simulink model "three_leg_switched"  (R2025b)
settings: Solver=FixedStepDiscrete  StartTime=0.0  StopTime=Tstop  FixedStep=Ts  RelTol=1e-3
values from neighbouring files (symbols this model uses):
  C = case_params(S, phase_deg, strcmp(policy, 'plan'), td_us, Ts)    [run_case.m]
  Tsw = C.Tsw    [ctrl_step.m]
undefined symbols (not defined in the file or in its folder): Ts
libraries: fl_lib x9, nesl_utility x8, ee_lib x6
settings Model: Creator=Asus ROG Strix G16  LastModifiedBy=Asus ROG Strix G16
settings DataIOCC: SaveOutput=off  SignalLogging=off  SaveTime=off

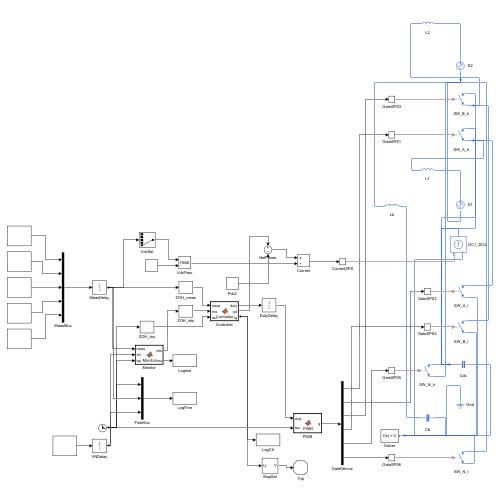
[thumbnail: Simulink's stored preview of the top-level diagram]
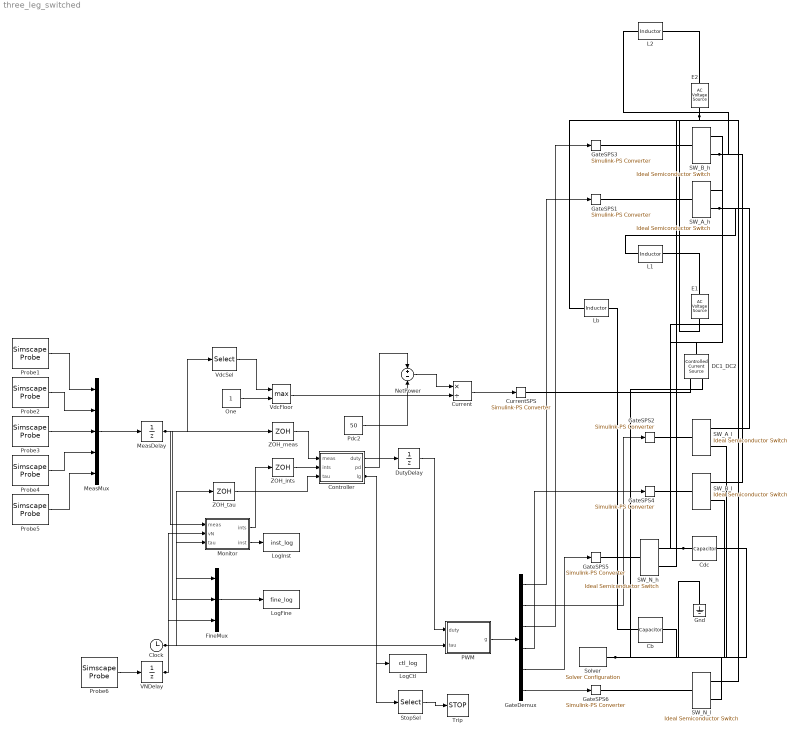
== system three_leg_switched ==
  Cb : fl_lib/Electrical/Electrical Elements/Capacitor  c=0.00025000000000000001 F  r=0 Ohm  g=0 1/Ohm  i_specify=off  i_priority=None  i=0 A  i_nominal_specify=off  i_nominal_value=1  i_nominal_unit=A  v_specify=off  v_priority=None  v=0 V  v_nominal_specify=off  v_nominal_value=1  v_nominal_unit=V  vc_specify=on  vc_priority=High  vc=C.vb0 V  vc_nominal_specify=off  vc_nominal_value=1  vc_nominal_unit=V
  Cdc : fl_lib/Electrical/Electrical Elements/Capacitor  c=2.0000000000000002e-05 F  r=0 Ohm  g=0 1/Ohm  i_specify=off  i_priority=None  i=0 A  i_nominal_specify=off  i_nominal_value=1  i_nominal_unit=A  v_specify=off  v_priority=None  v=0 V  v_nominal_specify=off  v_nominal_value=1  v_nominal_unit=V  vc_specify=on  vc_priority=High  vc=C.Vdc0 V  vc_nominal_specify=off  vc_nominal_value=1  vc_nominal_unit=V
  Clock : Clock
  Controller : MATLAB Function  TreatAsAtomicUnit=on
  Current : Product  Inputs=*/
  CurrentSPS : nesl_utility/Simulink-PS Converter  PhysicalDomain=network_engine_domain  SubClassName=ps_input  LeftPortType=input  RightPortType=output  PseudoPeriodic=off  Frequencies=[]  NoiseDistribution=none  NoiseParameters=[]  Unit=1  AffineConversion=off  FilteringAndDerivatives=provide  SimscapeFilterOrder=1  InputFilterTimeConstant=0.001  UdotUserProvided=0
  DC1_DC2 : fl_lib/Electrical/Electrical Sources/Controlled Current Source
  DutyDelay : UnitDelay  InitialCondition=C.duty0  SampleTime=Tsw  HasFrameUpgradeWarning=on
  E1 : fl_lib/Electrical/Electrical Sources/AC Voltage Source  amp=80 V  shift=C.theta0_deg deg  frequency=50 Hz
  E2 : fl_lib/Electrical/Electrical Sources/AC Voltage Source  amp=80 V  shift=C.theta0_deg + 0 deg  frequency=50 Hz
  FineMux : Mux  Inputs=3
  GateDemux : Demux  Outputs=6
  GateSPS{1..6} (6 alike) : nesl_utility/Simulink-PS Converter  PhysicalDomain=network_engine_domain  SubClassName=ps_input  LeftPortType=input  RightPortType=output  PseudoPeriodic=off  Frequencies=[]  NoiseDistribution=none  NoiseParameters=[]  Unit=1  AffineConversion=off  FilteringAndDerivatives=provide  SimscapeFilterOrder=1  InputFilterTimeConstant=0.001  UdotUserProvided=0
  Gnd : fl_lib/Electrical/Electrical Elements/Electrical Reference
  L1 : fl_lib/Electrical/Electrical Elements/Inductor  l=0.002 H  r=0.10000000000000001 Ohm  g=1e-9 1/Ohm  i_specify=off  i_priority=None  i=0 A  i_nominal_specify=off  i_nominal_value=1  i_nominal_unit=A  v_specify=off  v_priority=None  v=0 V  v_nominal_specify=off  v_nominal_value=1  v_nominal_unit=V  i_L_specify=on  i_L_priority=High  i_L=C.i10 A  i_L_nominal_specify=off  i_L_nominal_value=1  i_L_nominal_unit=A
  L2 : fl_lib/Electrical/Electrical Elements/Inductor  l=0.002 H  r=0.10000000000000001 Ohm  g=1e-9 1/Ohm  i_specify=off  i_priority=None  i=0 A  i_nominal_specify=off  i_nominal_value=1  i_nominal_unit=A  v_specify=off  v_priority=None  v=0 V  v_nominal_specify=off  v_nominal_value=1  v_nominal_unit=V  i_L_specify=on  i_L_priority=High  i_L=C.i20 A  i_L_nominal_specify=off  i_L_nominal_value=1  i_L_nominal_unit=A
  Lb : fl_lib/Electrical/Electrical Elements/Inductor  l=0.001 H  r=0.10000000000000001 Ohm  g=1e-9 1/Ohm  i_specify=off  i_priority=None  i=0 A  i_nominal_specify=off  i_nominal_value=1  i_nominal_unit=A  v_specify=off  v_priority=None  v=0 V  v_nominal_specify=off  v_nominal_value=1  v_nominal_unit=V  i_L_specify=on  i_L_priority=High  i_L=C.ib0 A  i_L_nominal_specify=off  i_L_nominal_value=1  i_L_nominal_unit=A
  LogCtl : ToWorkspace  VariableName=ctl_log  SampleTime=-1
  LogFine : ToWorkspace  VariableName=fine_log  SampleTime=-1
      settings: Decimation=fine_dec
  LogInst : ToWorkspace  VariableName=inst_log  SampleTime=-1
      settings: MaxDataPoints=1
  MeasDelay : UnitDelay  InitialCondition=C.meas0  SampleTime=Ts  HasFrameUpgradeWarning=on
  MeasMux : Mux  Inputs=5
  Monitor : MATLAB Function  TreatAsAtomicUnit=on
  NetPower : Sum  Inputs=+-
  One : Constant
  PWM : MATLAB Function  TreatAsAtomicUnit=on
  Pdc2 : Constant  Value=50
  Probe1 : SimscapeProbe  BoundBlock=7  Variables="{\"i_L\":{\"Probing\":\"ON\"}}"
  Probe2 : SimscapeProbe  BoundBlock=8  Variables="{\"i_L\":{\"Probing\":\"ON\"}}"
  Probe3 : SimscapeProbe  BoundBlock=6  Variables="{\"i_L\":{\"Probing\":\"ON\"}}"
  Probe4 : SimscapeProbe  BoundBlock=5  Variables="{\"vc\":{\"Probing\":\"ON\"}}"
  Probe5 : SimscapeProbe  BoundBlock=3  Variables="{\"vc\":{\"Probing\":\"ON\"}}"
  Probe6 : SimscapeProbe  BoundBlock=16  Variables="{\"v\":{\"Probing\":\"ON\"}}"
  SW_A_h : ee_lib/Semiconductors & Converters/Ideal Semiconductor Switch  port_option=ee.enum.controlport.ps  Ron=0.050000000000000003 Ohm  Goff=1e-6 1/Ohm  Vth=0.5 V  diode_param=ee.enum.converters.protectiondiode.nodynamics  diode_Vf=0.80000000000000004 V  diode_Ron=0.050000000000000003 Ohm  diode_Goff=1e-5 1/Ohm  diode_C=50e-9 F  diode_iRM=-235 A  diode_iF=300 A  diode_idot=-50 A/us  diode_trr_param=ee.enum.converters.diodetrr.trr_factor  diode_trr_factor=3  diode_trr=15 us  diode_Qrr=1500 s*uA
  SW_A_l : ee_lib/Semiconductors & Converters/Ideal Semiconductor Switch  port_option=ee.enum.controlport.ps  Ron=0.050000000000000003 Ohm  Goff=1e-6 1/Ohm  Vth=0.5 V  diode_param=ee.enum.converters.protectiondiode.nodynamics  diode_Vf=0.80000000000000004 V  diode_Ron=0.050000000000000003 Ohm  diode_Goff=1e-5 1/Ohm  diode_C=50e-9 F  diode_iRM=-235 A  diode_iF=300 A  diode_idot=-50 A/us  diode_trr_param=ee.enum.converters.diodetrr.trr_factor  diode_trr_factor=3  diode_trr=15 us  diode_Qrr=1500 s*uA
  SW_B_h : ee_lib/Semiconductors & Converters/Ideal Semiconductor Switch  port_option=ee.enum.controlport.ps  Ron=0.050000000000000003 Ohm  Goff=1e-6 1/Ohm  Vth=0.5 V  diode_param=ee.enum.converters.protectiondiode.nodynamics  diode_Vf=0.80000000000000004 V  diode_Ron=0.050000000000000003 Ohm  diode_Goff=1e-5 1/Ohm  diode_C=50e-9 F  diode_iRM=-235 A  diode_iF=300 A  diode_idot=-50 A/us  diode_trr_param=ee.enum.converters.diodetrr.trr_factor  diode_trr_factor=3  diode_trr=15 us  diode_Qrr=1500 s*uA
  SW_B_l : ee_lib/Semiconductors & Converters/Ideal Semiconductor Switch  port_option=ee.enum.controlport.ps  Ron=0.050000000000000003 Ohm  Goff=1e-6 1/Ohm  Vth=0.5 V  diode_param=ee.enum.converters.protectiondiode.nodynamics  diode_Vf=0.80000000000000004 V  diode_Ron=0.050000000000000003 Ohm  diode_Goff=1e-5 1/Ohm  diode_C=50e-9 F  diode_iRM=-235 A  diode_iF=300 A  diode_idot=-50 A/us  diode_trr_param=ee.enum.converters.diodetrr.trr_factor  diode_trr_factor=3  diode_trr=15 us  diode_Qrr=1500 s*uA
  SW_N_h : ee_lib/Semiconductors & Converters/Ideal Semiconductor Switch  port_option=ee.enum.controlport.ps  Ron=0.050000000000000003 Ohm  Goff=1e-6 1/Ohm  Vth=0.5 V  diode_param=ee.enum.converters.protectiondiode.nodynamics  diode_Vf=0.80000000000000004 V  diode_Ron=0.050000000000000003 Ohm  diode_Goff=1e-5 1/Ohm  diode_C=50e-9 F  diode_iRM=-235 A  diode_iF=300 A  diode_idot=-50 A/us  diode_trr_param=ee.enum.converters.diodetrr.trr_factor  diode_trr_factor=3  diode_trr=15 us  diode_Qrr=1500 s*uA
  SW_N_l : ee_lib/Semiconductors & Converters/Ideal Semiconductor Switch  port_option=ee.enum.controlport.ps  Ron=0.050000000000000003 Ohm  Goff=1e-6 1/Ohm  Vth=0.5 V  diode_param=ee.enum.converters.protectiondiode.nodynamics  diode_Vf=0.80000000000000004 V  diode_Ron=0.050000000000000003 Ohm  diode_Goff=1e-5 1/Ohm  diode_C=50e-9 F  diode_iRM=-235 A  diode_iF=300 A  diode_idot=-50 A/us  diode_trr_param=ee.enum.converters.diodetrr.trr_factor  diode_trr_factor=3  diode_trr=15 us  diode_Qrr=1500 s*uA
  Solver : nesl_utility/Solver Configuration  PhysicalDomain=network_engine_domain  SubClassName=solver  LeftPortType=input  RightPortType=generic  Tones=[]  Harmonics=[]  SimulateNoise=off  Profile=off  UseLocalSampling=off  EnableSwitchedLinearOptims=on  FrequencyDomain=off  UseCCode=off  RelTol=0.001  AbsTol=0.001  MinStep=1e-09  ToWorkspace=off  RevertToSquareIcSolve=off  NumHomotopyIterations=100  PhasorMode=off  PhasorModeNumHarmonics=1  ConsistencySolver=NEWTON_XTOL_AFTER_FTOL  IndexReductionMethod=DerivativeReplacement  DoDC=off  ResidualTolerance=1e-09  ConsistencyTolSource=GLOBAL  ConsistencyAbsTol=0.001  ConsistencyRelTol=0.001  ConsistencyTolFactor=0.001  UseLocalSolver=on  LocalSolverChoice=NE_PARTITIONING_ADVANCER  ResolveIndetEquations=on  FunctionEvalNumThread=1  LocalSolverSampleTime=Ts  DoFixedCost=on  MaxNonlinIter=3  MaxModeIter=2  ComputeImpulses=off  ImpulseIterations=2  LinearAlgebra=auto  LinearAlgebraNumThread=0  EquationFormulation=NE_TIME_EF  DelaysMemoryBudget=1024  AutomaticFiltering=on  FilteringTimeConstant=0.001  PartitionStorageMethod=AS_NEEDED  PartitionMemoryBudget=1024  PartitionMethod=ROBUST  MultibodyUseLocalSolver=off  MultibodyLocalSolverChoice=ODE1  MultibodyLocalSolverSampleTime=0.001
  StopSel : Selector  InputPortWidth=27  IndexOptions=Index vector (dialog)  Indices=27  OutputSizes=1
  Trip : Stop
  VNDelay : UnitDelay  InitialCondition=C.vb0  SampleTime=Ts  HasFrameUpgradeWarning=on
  VdcFloor : MinMax  Function=max  Inputs=2
  VdcSel : Selector  InputPortWidth=5  IndexOptions=Index vector (dialog)  Indices=5  OutputSizes=1
  ZOH_ints : ZeroOrderHold  SampleTime=Tsw
  ZOH_meas : ZeroOrderHold  SampleTime=Tsw
  ZOH_tau : ZeroOrderHold  SampleTime=Tsw
  wires:
  Probe5/1 -> MeasMux/5
  Probe1/1 -> MeasMux/1
  Probe6/1 -> VNDelay/1
  One/1 -> VdcFloor/2
  MeasMux/1 -> MeasDelay/1
  GateDemux/2 -> GateSPS2/1
  Probe2/1 -> MeasMux/2
  MeasDelay/1 -> ZOH_meas/1, Monitor/1(meas), VdcSel/1, FineMux/2
  PWM/1(g) -> GateDemux/1
  Probe3/1 -> MeasMux/3
  Probe4/1 -> MeasMux/4
  Clock/1 -> ZOH_tau/1, Monitor/3(tau), PWM/2(tau), FineMux/1
  VNDelay/1 -> Monitor/2(vN), FineMux/3
  VdcSel/1 -> VdcFloor/1
  ZOH_tau/1 -> Controller/3(tau)
  Monitor/1(ints) -> ZOH_ints/1
  Monitor/2(inst) -> LogInst/1
  FineMux/1 -> LogFine/1
  VdcFloor/1 -> Current/2
  ZOH_meas/1 -> Controller/1(meas)
  ZOH_ints/1 -> Controller/2(ints)
  NetPower/1 -> Current/1
  Pdc2/1 -> NetPower/2
  Controller/1(duty) -> DutyDelay/1
  DutyDelay/1 -> PWM/1(duty)
  Controller/2(pd) -> NetPower/1
  Controller/3(lg) -> LogCtl/1, StopSel/1
  GateDemux/1 -> GateSPS1/1
  StopSel/1 -> Trip/1
  Current/1 -> CurrentSPS/1
  GateDemux/3 -> GateSPS3/1
  GateDemux/4 -> GateSPS4/1
  GateDemux/5 -> GateSPS5/1
  GateDemux/6 -> GateSPS6/1
  connections:
  Lb/RConn1 -- Cb/LConn1
  GateSPS6/RConn1 -- SW_N_l/LConn1
  L2/RConn1 -- E2/LConn1
  GateSPS5/RConn1 -- SW_N_h/LConn1
  GateSPS2/RConn1 -- SW_A_l/LConn1
  CurrentSPS/RConn1 -- DC1_DC2/RConn1
  GateSPS1/RConn1 -- SW_A_h/LConn1
  SW_N_h/RConn1 -- DC1_DC2/LConn1 -- SW_A_h/RConn1 -- SW_B_h/RConn1 -- Cdc/LConn1
  Lb/LConn1 -- E1/RConn1 -- E2/RConn1 -- SW_N_l/RConn1 -- SW_N_h/RConn2
  GateSPS3/RConn1 -- SW_B_h/LConn1
  L2/LConn1 -- SW_B_l/RConn1 -- SW_B_h/RConn2
  L1/LConn1 -- SW_A_l/RConn1 -- SW_A_h/RConn2
  GateSPS4/RConn1 -- SW_B_l/LConn1
  L1/RConn1 -- E1/LConn1
  Cb/RConn1 -- DC1_DC2/RConn2 -- SW_N_l/RConn2 -- Cdc/RConn1 -- SW_A_l/RConn2 -- SW_B_l/RConn2 -- Solver/RConn1 -- Gnd/LConn1

== matlab function three_leg_switched/Controller ==
  data: meas input; duty output; ints input; tau input; pd output; lg output; C parameter
function [duty, pd, lg] = Controller(meas, ints, tau, C)
%#codegen
[duty, pd, lg] = ctrl_step(meas, ints, tau, C);

== matlab function three_leg_switched/Monitor ==
  data: meas input; ints output; vN input; tau input; inst output; C parameter
function [ints, inst] = Monitor(meas, vN, tau, C)
%#codegen
[ints, inst] = fine_monitor(meas, vN, tau, C);

== matlab function three_leg_switched/PWM ==
  data: duty input; g output; tau input; C parameter
function g = PWM(duty, tau, C)
%#codegen
g = pwm_gates(duty, tau, C);
